simulink model "simulinkACTC"  (R2019a)
settings: Solver=VariableStepAuto  StartTime=0.0  StopTime=10  RelTol=1e-3
values from neighbouring files (symbols this model uses):
  A = [5.0; 5.0; 0.5]    [SCARA_Init.m]
  B = [0.5; 0.5; 0.02]    [SCARA_Init.m]
  C = [27.5; 27.5; 0.7]    [SCARA_Init.m]
  f = [0.01; 0.01; 0.05]    [SCARA_Init.m]
  g_vec = [0, 0, -g, 0]    [SCARA_Init.m]
  J1 = [ (1/6)*m1*L1^2, 0, 0, m1*(L1/2) ... (first row only)    [SCARA_Init.m]
  J2 = [ (1/6)*m2*L2^2, 0, 0, m2*(L2/2) ... (first row only)    [SCARA_Init.m]
  L1 = 0.45    [SCARA_Init.m]
  L2 = 0.35    [SCARA_Init.m]
  L3 = 0.5    [SCARA_Init.m]
  m1 = 14    [SCARA_Init.m]
  m2 = 18    [SCARA_Init.m]
  m3 = 2    [SCARA_Init.m]
  r = 0.02    [SCARA_Init.m]
  rc1 = [L1/2; 0; 0; 1]    [SCARA_Init.m]
  rc2 = [L2/2; 0; 0; 1]    [SCARA_Init.m]
settings Model: Creator=bahaa  LastModifiedBy=bahaa

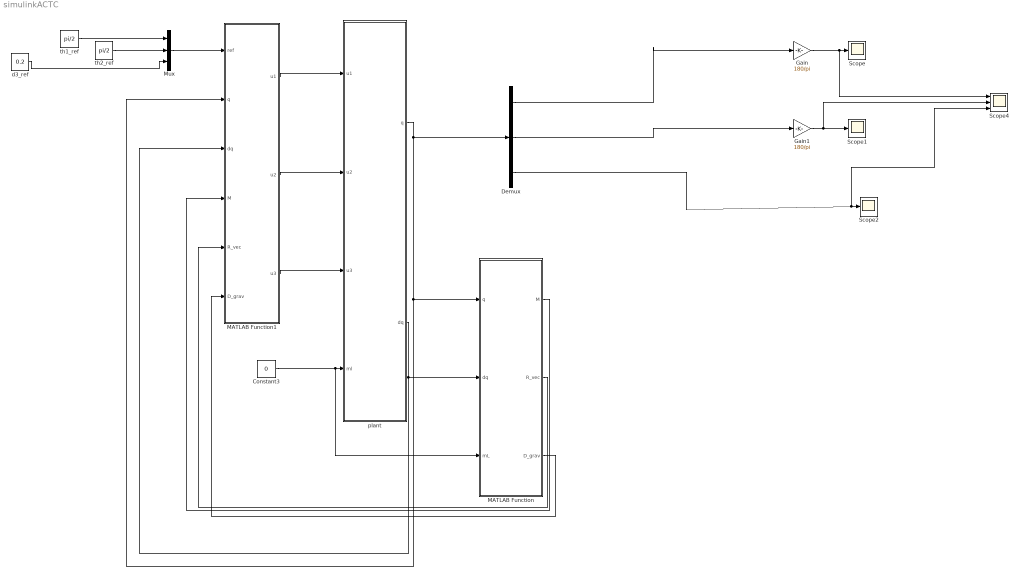
== system simulinkACTC ==
  Constant3 : Constant  Value=0
  Demux : Demux  Outputs=3
  Gain : Gain  Gain=180/pi
  Gain1 : Gain  Gain=180/pi
  MATLAB Function : MATLAB Function  TreatAsAtomicUnit=on
  MATLAB Function1 : MATLAB Function  TreatAsAtomicUnit=on  SystemSampleTime=0.001
  Mux : Mux  Inputs=3
  Scope : Scope
  Scope1 : Scope
  Scope2 : Scope
  Scope4 : Scope  NumInputPorts=3
  d3_ref : Constant  Value=0.2
  plant : Subsystem
  th1_ref : Constant  Value=pi/2
  th2_ref : Constant  Value=pi/2
  wires:
  MATLAB Function/3(D_grav) -> MATLAB Function1/6(D_grav)
  th2_ref/1 -> Mux/2
  Gain/1 -> Scope4/1, Scope/1
  Demux/2 -> Gain1/1
  Mux/1 -> MATLAB Function1/1(ref)
  plant/2(dq) -> MATLAB Function1/3(dq), MATLAB Function/2(dq)
  MATLAB Function/2(R_vec) -> MATLAB Function1/5(R_vec)
  Demux/1 -> Gain/1
  MATLAB Function1/1(u1) -> plant/1(u1)
  MATLAB Function/1(M) -> MATLAB Function1/4(M)
  Constant3/1 -> MATLAB Function/3(mL), plant/4(ml)
  Demux/3 -> Scope4/3, Scope2/1
  plant/1(q) -> Demux/1, MATLAB Function1/2(q), MATLAB Function/1(q)
  th1_ref/1 -> Mux/1
  MATLAB Function1/2(u2) -> plant/2(u2)
  d3_ref/1 -> Mux/3
  Gain1/1 -> Scope4/2, Scope1/1
  MATLAB Function1/3(u3) -> plant/3(u3)

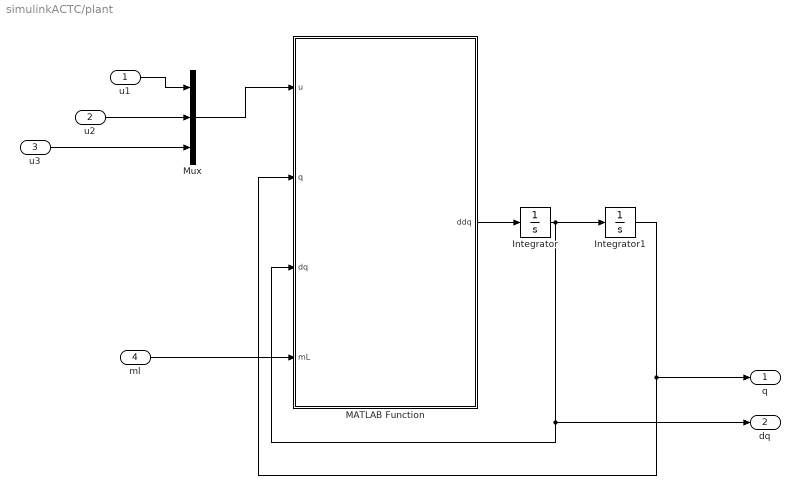
== system simulinkACTC/plant ==
  u1 : Inport
  u2 : Inport  Port=2
  u3 : Inport  Port=3
  ml : Inport  Port=4
  Integrator : Integrator  InitialCondition=[0;0;0]
  Integrator1 : Integrator  InitialCondition=[0;0;0]
  MATLAB Function : MATLAB Function  TreatAsAtomicUnit=on
  Mux : Mux  Inputs=3
  q : Outport
  dq : Outport  Port=2
  wires:
  Integrator1/1 -> q/1, MATLAB Function/2(q)
  MATLAB Function/1(ddq) -> Integrator/1
  Mux/1 -> MATLAB Function/1(u)
  Integrator/1 -> MATLAB Function/3(dq), dq/1, Integrator1/1
  u2/1 -> Mux/2
  ml/1 -> MATLAB Function/4(mL)
  u1/1 -> Mux/1
  u3/1 -> Mux/3

== matlab function simulinkACTC/MATLAB Function1 ==
  data: ref input; u1 output; q input; dq input; M input; R_vec input; D_grav input; u2 output; u3 output; A parameter
function [u1, u2, u3] = scara_regressor_actc(ref, q, dq, M, R_vec, D_grav, A)

    dt = 0.001; % خطوة المحاكاة


  %الذاكرة 
    persistent theta1 theta2 theta3;
    
    
    theta_nom = [1; 1; 1; 0]; 

    if isempty(theta1)
        theta1 = theta_nom;
        theta2 = theta_nom;
        theta3 = theta_nom;
    end


    Lambda = diag([50, 50, 50]);     % ميل سطح الانزلاق
    
    Ks = [100; 100; 100];              
    %هذا الثابت مضروب بديناميكية الخطا ليحذه ريثما يتم تقدير بارامترات تكيفية جيدة تجعل النظام مستقر
    %بالمختصر يعوض التاخير الزمني في عملية التقدير 
    
    
%سرعة التكيف
    Gamma = diag([10, 10, 10, 10]);     
    
    sigma = 0.01;                  %هذا الثابت يمنع البارامترات من الابتعاد كثيراً عن النموذج الاساسي
%حساب الاخطاء
    e = ref - q;
    
    dq_ref = [0; 0; 0];
    ddq_ref = [0; 0; 0];
    de = dq_ref - dq;

    s = de + Lambda * e;

 % حساب التسارع المرجعي
    ddq_r = ddq_ref + Lambda * de;

%البارامترات المقدرة الخاصة بكل حد
    Tau_M = M * ddq_r;    % عزم العطالة
    Tau_V = R_vec;        %الاحتكاك مع ثوابت حدود اخرى
    Tau_G = D_grav;       % عزم الجاذبية

%تطبيق قانون تحديث البارامترات 
    Tau_total = zeros(3,1);
    
%المفصل الاول 
    % بناء شعاع الانحدار Y
    Y1 = [Tau_M(1); Tau_V(1); Tau_G(1); 1]; 
    
    % قانون التحديث 
    dtheta1 = (Gamma * Y1 * s(1)) / (1 + Y1' * Y1) - sigma * (theta1 - theta_nom);
    theta1 = theta1 + dtheta1 * dt;
    
    % قانون التحكم 
    Tau_total(1) = theta1' * Y1 + Ks(1) * s(1);

    %المفصل الثاني 
    Y2 = [Tau_M(2); Tau_V(2); Tau_G(2); 1]; 
    
    dtheta2 = (Gamma * Y2 * s(2)) / (1 + Y2' * Y2) - sigma * (theta2 - theta_nom);
    theta2 = theta2 + dtheta2 * dt;
    
    Tau_total(2) = theta2' * Y2 + Ks(2) * s(2);

     % Joint 3 
    Y3 = [Tau_M(3); Tau_V(3); Tau_G(3); 1]; 
    
    dtheta3 = (Gamma * Y3 * s(3)) / (1 + Y3' * Y3) - sigma * (theta3 - theta_nom);
    theta3 = theta3 + dtheta3 * dt;
    
    Tau_total(3) = theta3' * Y3 + Ks(3) * s(3);

%تحويل العزم لجهد
    A_matrix = diag(A);
    u_total = A_matrix \ Tau_total; 

  
    u1 = u_total(1);
    u2 = u_total(2);
    u3 = u_total(3);
end

== matlab function simulinkACTC/plant/MATLAB Function ==
  data: u input; ddq output; q input; dq input; mL input; g_vec parameter; f parameter; C parameter; B parameter; A parameter; J2 parameter; J1 parameter; rc2 parameter; rc1 parameter; m3 parameter; m2 parameter; m1 parameter; r parameter; L3 parameter; L2 parameter; L1 parameter
function ddq = scara_plant_numerical(u, q, dq, mL, g_vec, f, C, B, A, J2, J1, rc2, rc1, m3, m2, m1, r, L3, L2, L1)
    
    %المداخل المتغيرة u q dq mL
  
    %الزوايا
    th1 = q(1); 
    th2 = q(2);
    d3  = q(3);

%حساب كل المتغيرات التي تعتمد على تغير الحمل mL
    m3_star = m3 + mL;%كتلة الوصلة الثالثة بعد اضافة الحمل 
    zc3_star = (m3*(L3/2) + mL*L3) / m3_star;
    rc3 = [0; 0; -zc3_star; 1]; %مركز الثقل الجديد للوصلة الثالثة بعد اضافة الحمل 
    
    h3 = abs(zc3_star - (L3/2));%الازاحة بين مركز الثقل القديم والجديد للوصلة
    hL = abs(L3 - zc3_star);%الازاحة  للححمل 
    I_xx3_star = (1/12)*m3*L3^2 + m3*h3^2 + mL*hL^2;
    
    % مصفوفة J3
    J3 = [ (1/2)*m3*r^2, 0, 0, 0;
           0, (1/2)*m3*r^2, 0, 0;
           0, 0, (2*I_xx3_star - (1/2)*m3*r^2), -m3_star*zc3_star;
           0, 0, -m3_star*zc3_star, m3_star ];


    % حساب Uij
   
    A1 = [cos(th1), -sin(th1), 0, L1*cos(th1);
          sin(th1),  cos(th1), 0, L1*sin(th1);
          0,         0,        1, 0;
          0,         0,        0, 1];

    A2 = [cos(th2),  sin(th2), 0, L2*cos(th2);
          sin(th2), -cos(th2), 0, L2*sin(th2);
          0,         0,       -1, 0;
          0,         0,        0, 1];

    A3 = [1, 0, 0, 0;
          0, 1, 0, 0;
          0, 0, 1, d3;
          0, 0, 0, 1];

    
    T01 = A1;
    T02 = T01 * A2;
    T03 = T02 * A3;

    
    %الدوراني 
    Q_rev = [0, -1, 0, 0;
             1,  0, 0, 0;
             0,  0, 0, 0;
             0,  0, 0, 0];
   %الانسحابي
    Q_pris = [0, 0, 0, 0;
              0, 0, 0, 0;
              0, 0, 0, 1;
              0, 0, 0, 0];

    U11 = Q_rev * T01;
    U12 = Q_rev * T02;
    U13 = Q_rev * T03;   
    U22 = T01 * Q_rev * A2;
    U23 = T01 * Q_rev * (A2 * A3);
    U33 = T02 * Q_pris * A3;

%Dij حساب 
    D11 = trace(U11*J1*U11') + trace(U12*J2*U12') + trace(U13*J3*U13');
    D12 = trace(U12*J2*U22') + trace(U13*J3*U23'); 
    D21 = D12; % المصفوفة متناظرة
    D22 = trace(U22*J2*U22') + trace(U23*J3*U23');
    D33 = trace(U33*J3*U33');

%حساب Di 
    D_grav = zeros(3,1);
    D_grav(1) = -m1*(g_vec * U11 * rc1) - m2*(g_vec * U12 * rc2) - m3_star*(g_vec * U13 * rc3);
    D_grav(2) = -m2*(g_vec * U22 * rc2) - m3_star*(g_vec * U23 * rc3);
    D_grav(3) = -m3_star*(g_vec * U33 * rc3);

% هذه المصفوفة حصلنا عليها بعد ان عزلنا اعلى مشتق
    M = zeros(3,3);
    M(1,1) = D11 + B(1);
    M(1,2) = D12;
    M(2,1) = D21;
    M(2,2) = D22 + B(2);
    M(3,3) = D33 + B(3);

    R_vec = zeros(3,1);
    R_vec(1) = (f(1) + C(1)) * dq(1);
    R_vec(2) = (f(2) + C(2)) * dq(2);
    R_vec(3) = (f(3) + C(3)) * dq(3);

    Tau_actuator = [A(1)*u(1); A(2)*u(2); A(3)*u(3)];
    RHS = Tau_actuator - R_vec - D_grav;

    ddq = M \ RHS; % حساب أعلى مشتق
end

== matlab function simulinkACTC/MATLAB Function ==
  data: q input; M output; dq input; mL input; R_vec output; D_grav output; L1 parameter; L2 parameter; L3 parameter; r parameter; m1 parameter; m2 parameter; m3 parameter; rc1 parameter; rc2 parameter; J1 parameter; J2 parameter; B parameter; C parameter; f parameter; g_vec parameter
function [M, R_vec, D_grav] = scara_dynamics_estimator(q, dq, mL, L1, L2, L3, r, m1, m2, m3, rc1, rc2, J1, J2, B, C, f, g_vec)

    th1 = q(1); 
    th2 = q(2);
    d3  = q(3);
    
    % 2. المتغيرات المعتمدة على الحمل (mL)
    m3_star = m3 + mL;
    zc3_star = (m3*(L3/2) + mL*L3) / m3_star;
    rc3 = [0; 0; -zc3_star; 1]; 
    
    h3 = abs(zc3_star - (L3/2));
    hL = abs(L3 - zc3_star);
    I_xx3_star = (1/12)*m3*L3^2 + m3*h3^2 + mL*hL^2;
    
    J3 = [ (1/2)*m3*r^2, 0, 0, 0;
           0, (1/2)*m3*r^2, 0, 0;
           0, 0, (2*I_xx3_star - (1/2)*m3*r^2), -m3_star*zc3_star;
           0, 0, -m3_star*zc3_star, m3_star ];

    % 3. مصفوفات التحويل والمشتقات (Uij)
    A1 = [cos(th1), -sin(th1), 0, L1*cos(th1); sin(th1), cos(th1), 0, L1*sin(th1); 0, 0, 1, 0; 0, 0, 0, 1];
    A2 = [cos(th2), sin(th2), 0, L2*cos(th2); sin(th2), -cos(th2), 0, L2*sin(th2); 0, 0, -1, 0; 0, 0, 0, 1];
    A3 = [1, 0, 0, 0; 0, 1, 0, 0; 0, 0, 1, d3; 0, 0, 0, 1];

    T01 = A1; T02 = T01 * A2; T03 = T02 * A3;

    Q_rev = [0, -1, 0, 0; 1, 0, 0, 0; 0, 0, 0, 0; 0, 0, 0, 0];
    Q_pris = [0, 0, 0, 0; 0, 0, 0, 0; 0, 0, 0, 1; 0, 0, 0, 0];

    U11 = Q_rev * T01; U12 = Q_rev * T02; U13 = Q_rev * T03;   
    U22 = T01 * Q_rev * A2; U23 = T01 * Q_rev * (A2 * A3); U33 = T02 * Q_pris * A3;

    % 4. حساب مصفوفة العطالة (M)
    D11 = trace(U11*J1*U11') + trace(U12*J2*U12') + trace(U13*J3*U13');
    D12 = trace(U12*J2*U22') + trace(U13*J3*U23'); 
    D21 = D12; 
    D22 = trace(U22*J2*U22') + trace(U23*J3*U23'); 
    D33 = trace(U33*J3*U33');

    M = zeros(3,3);
    M(1,1) = D11 + B(1); M(1,2) = D12; M(2,1) = D21; M(2,2) = D22 + B(2); M(3,3) = D33 + B(3);

    % 5. حساب شعاع الجاذبية (D_grav)
    D_grav = zeros(3,1);
    D_grav(1) = -m1*(g_vec * U11 * rc1) - m2*(g_vec * U12 * rc2) - m3_star*(g_vec * U13 * rc3);
    D_grav(2) = -m2*(g_vec * U22 * rc2) - m3_star*(g_vec * U23 * rc3);
    D_grav(3) = -m3_star*(g_vec * U33 * rc3);

    % 6. حساب شعاع الاحتكاك (R_vec)
    R_vec = zeros(3,1);
    R_vec(1) = (f(1) + C(1)) * dq(1); 
    R_vec(2) = (f(2) + C(2)) * dq(2); 
    R_vec(3) = (f(3) + C(3)) * dq(3);
end
